simulink model "example_sim_airfoilDynStall"  (R2018b)
settings: Solver=FixedStepAuto  StartTime=0.0  StopTime=t_sim  FixedStep=0.002  RelTol=1e-3
values from neighbouring files (symbols this model uses):
  a = 300    [example_airfoilDynStall.m]
  alpha_0 = 4    [example_airfoilDynStall.m]
  c = 2.8    [example_airfoilDynStall.m]
  Delta_alpha = alpha-alpha0    [airfoilDynStallClFs.m]    (also in example_airfoilDynStall.m = 5)
  fcd = airfoilAnalytic0515Ma( F15.wcd, Ma, F15.ncd, F15.ocd )    [example_airfoilDynStall.m]
  fcl = airfoilAnalytic0515Ma( F15.wcl, Ma, F15.ncl, F15.ocl )    [example_airfoilDynStall.m]
  fcm = airfoilAnalytic0515Ma( F15.wcm, Ma, F15.ncm, F15.ocm )    [example_airfoilDynStall.m]
  k = 0.075    [example_airfoilDynStall.m]
  V = Ma*a    (= 223.5)    [example_airfoilDynStall.m]
libraries: linear_systems_lib x2
settings Model: Creator=Ybeyer  LastModifiedBy=yannic

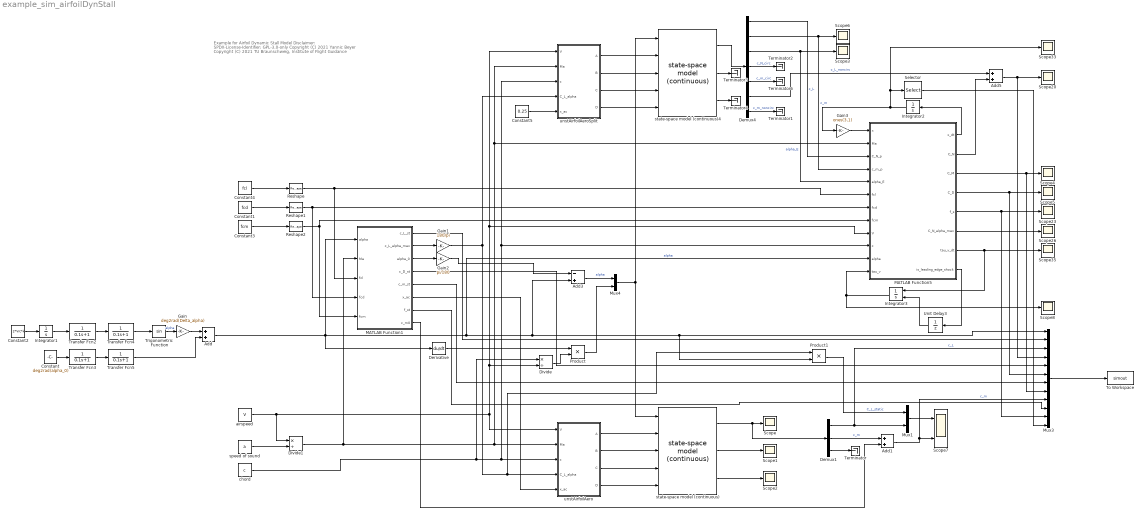
== system example_sim_airfoilDynStall ==
  note: Example for Airfoil Dynamic Stall Model
      |
      | Disclaimer:
      | SPDX-License-Identifier: GPL-3.0-only
      |
      | Copyright (C) 2021 Yannic Beyer
      | Copyright (C) 2021 TU Braunschweig, Institute of Flight Guidance
  Add : Sum
  Add1 : Sum
  Add3 : Sum  Inputs=-+
  Add5 : Sum
  Constant : Constant  Value=deg2rad(alpha_0)
  Constant1 : Constant  Value=fcd
  Constant2 : Constant  Value=2*V/c*k
  Constant3 : Constant  Value=fcm
  Constant4 : Constant  Value=fcl
  Constant5 : Constant  Value=0.25
  Demux1 : Demux  Outputs=3
  Demux4 : Demux  Outputs=7
  Derivative : Derivative
  Divide : Product  Inputs=*/
  Divide1 : Product  Inputs=*/
  Gain : Gain  Gain=deg2rad(Delta_alpha)
  Gain1 : Gain  Gain=180/pi
  Gain2 : Gain  Gain=pi/180
  Gain3 : Gain  Gain=ones(3,1)
  Integrator1 : Integrator
  Integrator2 : Integrator
  Integrator3 : Integrator  ExternalReset=falling
  MATLAB Function1 : MATLAB Function  TreatAsAtomicUnit=on
  MATLAB Function5 : MATLAB Function  TreatAsAtomicUnit=on
  Mux1 : Mux  Inputs=2
  Mux3 : Mux  Inputs=12
  Mux4 : Mux  Inputs=2
  Product : Product
  Product1 : Product
  Reshape : Reshape  OutputDimensionality=Row vector (2-D)
  Reshape1 : Reshape  OutputDimensionality=Row vector (2-D)
  Reshape2 : Reshape  OutputDimensionality=Row vector (2-D)
  Scope{,1..6,8,20,23,26,33,35} (13 alike) : Scope
  Scope7 : Scope  NumInputPorts=2
  Selector : Selector  InputPortWidth=3  IndexOptions=Index vector (dialog)  Indices=2  OutputSizes=1
  Terminator{,1..4,6} (6 alike) : Terminator
  To Workspace : ToWorkspace  VariableName=simout  SaveFormat=Timeseries  SampleTime=-1
  Transfer Fcn{2..5} (4 alike) : TransferFcn  Denominator=[0.1 1]
  Trigonometric Function : Trigonometry
  Unit Delay3 : UnitDelay  SampleTime=-1
  airspeed : Constant  Value=V
  chord : Constant  Value=c
  speed of sound : Constant  Value=a
  state-space model (continuous) : linear_systems_lib/state-space model  (continuous)
      settings: SourceProductName=LADAC
  state-space model (continuous)4 : linear_systems_lib/state-space model  (continuous)
      settings: SourceProductName=LADAC
  unstAirfoilAero : MATLAB Function  TreatAsAtomicUnit=on
  unstAirfoilAeroSplit : MATLAB Function  TreatAsAtomicUnit=on
  wires:
  unstAirfoilAero/4(D) -> state-space model (continuous)/5
  unstAirfoilAero/3(C) -> state-space model (continuous)/4
  unstAirfoilAero/2(B) -> state-space model (continuous)/3
  unstAirfoilAero/1(A) -> state-space model (continuous)/2
  chord/1 -> unstAirfoilAeroSplit/3(c), MATLAB Function5/10(c), unstAirfoilAero/3(c), Divide/1
  Mux4/1 -> state-space model (continuous)/1, state-space model (continuous)4/1
  state-space model (continuous)/1 -> Demux1/1, Scope/1
  state-space model (continuous)/2 -> Scope1/1
  state-space model (continuous)/3 -> Scope2/1
  Divide/1 -> Product/2
  Product/1 -> Mux4/2
  Demux1/1 -> Mux3/3, Mux1/2  "c_L"
  Add1/1 -> Mux3/9, Scope7/2  "c_m"
  Mux1/1 -> Scope7/1
  speed of sound/1 -> Divide1/2
  Derivative/1 -> Product/1
  Add/1 -> MATLAB Function5/11(alpha), Add3/2, Product1/2, Mux3/1, Derivative/1, MATLAB Function1/1(alpha)  "alpha"
  Product1/1 -> Mux1/1  "C_L_static"
  Mux3/1 -> To Workspace/1
  Trigonometric Function/1 -> Gain/1  "alpha"
  MATLAB Function1/1(c_L_st) -> Mux3/2
  Constant/1 -> Transfer Fcn3/1
  Gain/1 -> Add/1
  Transfer Fcn3/1 -> Transfer Fcn5/1
  Transfer Fcn2/1 -> Transfer Fcn4/1
  Integrator1/1 -> Transfer Fcn2/1
  Constant2/1 -> Integrator1/1
  Transfer Fcn4/1 -> Trigonometric Function/1
  Transfer Fcn5/1 -> Add/2
  Constant4/1 -> Reshape/1
  Add3/1 -> Mux4/1  "alpha"
  MATLAB Function1/3(alpha_0) -> Gain2/1
  Gain1/1 -> unstAirfoilAero/4(C_L_alpha), Product1/1, unstAirfoilAeroSplit/4(C_L_alpha)
  Gain2/1 -> Add3/1
  MATLAB Function5/1(x_dt) -> Integrator2/1
  Integrator2/1 -> Scope33/1, Selector/1, Gain3/1
  Divide1/1 -> unstAirfoilAeroSplit/2(Ma), MATLAB Function5/2(Ma), unstAirfoilAero/2(Ma), MATLAB Function1/2(Ma)
  Add5/1 -> Scope20/1, Mux3/4
  Gain3/1 -> MATLAB Function5/1(x)
  MATLAB Function5/6(C_N_alpha_max) -> Scope26/1
  state-space model (continuous)4/1 -> Demux4/1
  Demux4/6 -> Add5/1  "c_L_noncirc"
  unstAirfoilAeroSplit/4(D) -> state-space model (continuous)4/5
  unstAirfoilAeroSplit/3(C) -> state-space model (continuous)4/4
  unstAirfoilAeroSplit/2(B) -> state-space model (continuous)4/3
  unstAirfoilAeroSplit/1(A) -> state-space model (continuous)4/2
  airspeed/1 -> unstAirfoilAero/1(V), unstAirfoilAeroSplit/1(V), MATLAB Function5/9(V), Divide/2, Divide1/1
  MATLAB Function1/6(x_ac) -> unstAirfoilAero/5(x_ac)
  MATLAB Function5/5(f_s) -> Mux3/11, Scope23/1
  Reshape/1 -> MATLAB Function1/3(fcl), MATLAB Function5/6(fcl)
  MATLAB Function5/2(C_N) -> Add5/2
  MATLAB Function5/7(tau_v_dt) -> Scope35/1, Integrator3/1
  MATLAB Function5/8(is_leading_edge_shock) -> Unit Delay3/1
  Integrator3/1 -> MATLAB Function5/12(tau_v), Scope8/1
  Unit Delay3/1 -> Integrator3/2
  MATLAB Function1/2(c_L_alpha_max) -> Gain1/1
  state-space model (continuous)4/2 -> Terminator3/1
  state-space model (continuous)4/3 -> Terminator4/1
  Demux4/5 -> Terminator6/1  "c_m_circ"
  MATLAB Function5/3(C_M) -> Mux3/8, Scope4/1
  MATLAB Function5/4(C_D) -> Mux3/6, Scope5/1
  Demux4/3 -> Scope3/1, MATLAB Function5/5(alpha_E)  "alpha_E"
  Demux4/2 -> MATLAB Function5/4(c_m_p), Scope6/1  "c_m"
  Demux4/1 -> MATLAB Function5/3(C_N_p)  "c_L"
  Demux1/3 -> Terminator/1
  Constant1/1 -> Reshape1/1
  Constant3/1 -> Reshape2/1
  Reshape1/1 -> MATLAB Function1/4(fcd), MATLAB Function5/7(fcd)
  Reshape2/1 -> MATLAB Function5/8(fcm), MATLAB Function1/5(fcm)
  MATLAB Function1/4(c_D_st) -> Mux3/5
  MATLAB Function1/5(c_m_st) -> Mux3/7
  MATLAB Function1/7(f_st) -> Mux3/10
  Demux4/7 -> Terminator1/1  "c_m_noncirc"
  Selector/1 -> Mux3/12
  Demux4/4 -> Terminator2/1  "c_N_circ"
  Constant5/1 -> unstAirfoilAeroSplit/5(x_ac)
  Demux1/2 -> Add1/1  "c_m"
  MATLAB Function1/8(c_m0) -> Add1/2

== matlab function example_sim_airfoilDynStall/unstAirfoilAero ==
  data: V input; A output; Ma input; c input; C_L_alpha input; x_ac input; B output; C output; D output
function [A,B,C,D] = fcn( V, Ma, c, C_L_alpha, x_ac ) %#codegen
[A,B,C,D] = unstAirfoilAero( V, Ma, c, C_L_alpha, x_ac );
end

== matlab function example_sim_airfoilDynStall/MATLAB Function1 ==
  data: c_L_st output; alpha input; c_L_alpha_max output; Ma input; fcl input; alpha_0 output; fcd input; c_D_st output; c_m_st output; fcm input; x_ac output; f_st output; c_m0 output
function [c_L_st,c_L_alpha_max,alpha_0,c_D_st,c_m_st,x_ac,f_st,c_m0] = fcn(alpha,Ma, fcl,fcd, fcm)
alpha_deg = rad2deg(alpha);

c_L_st = airfoilAnalytic0515AlCl( fcl, grid2Coordinates( alpha_deg, Ma ) );
[C_N_alpha_max,alpha_0] = airfoilAnalytic0515ClAlphaMax( fcl, Ma );
c_L_alpha_max = C_N_alpha_max;

c_D_st = airfoilAnalytic0515AlCd( fcd, rad2deg(alpha) );

f_st = airfoilDynStallFst( c_L_st, c_L_alpha_max, alpha_deg-alpha_0 );
c_m_st = airfoilAnalyticBlCm( fcm, f_st, c_L_st );

x_ac = airfoilAnalyticBlXac( fcm );

c_m0 = airfoilAnalyticBlCm0( fcm );

end

== matlab function example_sim_airfoilDynStall/MATLAB Function5 ==
  data: x input; x_dt output; Ma input; C_N_p input; c_m_p input; alpha_E input; C_N output; C_M output; C_D output; fcl input; fcd input; fcm input; f_s output; V input; c input; C_N_alpha_max output; alpha input; tau_v input; tau_v_dt output; is_leading_edge_shock output
function [ x_dt, C_N, C_M, C_D, f_s, C_N_alpha_max, tau_v_dt, is_leading_edge_shock ] = airfoilDynStall( x, Ma, C_N_p, c_m_p, alpha_E, fcl, fcd, fcm, V, c, alpha, tau_v) %#codegen
[ x_dt, C_N, C_M, C_D, f_s, C_N_alpha_max, tau_v_dt, is_leading_edge_shock ] = airfoilDynStall( x, Ma, C_N_p, c_m_p, alpha_E, fcl, fcd, fcm, V, c, alpha, tau_v );
end

== matlab function example_sim_airfoilDynStall/unstAirfoilAeroSplit ==
  data: V input; A output; Ma input; c input; C_L_alpha input; x_ac input; B output; C output; D output
function [A,B,C,D] = fcn( V, Ma, c, C_L_alpha, x_ac ) %#codegen
[A,B,C,D] = unstAirfoilAeroSplit( V, Ma, c, C_L_alpha, x_ac );
end
